simulink subsystem "pendulum_nonlinear"  (R2024b)
settings: Solver=VariableStepAuto  StartTime=0.0  StopTime=10.0  RelTol=1e-3
undefined symbols (not defined in the file): params
settings Model: Creator=dsagn  LastModifiedBy=dsagn
settings ModelReferenceCC: UpdateModelReferenceTargets=IfOutOfDate
settings SFSimCC: SimGPUStackLimitPerThread=51200
settings RTWCC: GPUStackLimitPerThread=51200  GPUComputeCapability=7.5
settings ConfigComp: CovMetricSettings=de  CovBoundaryAbsTol=1.0e-5

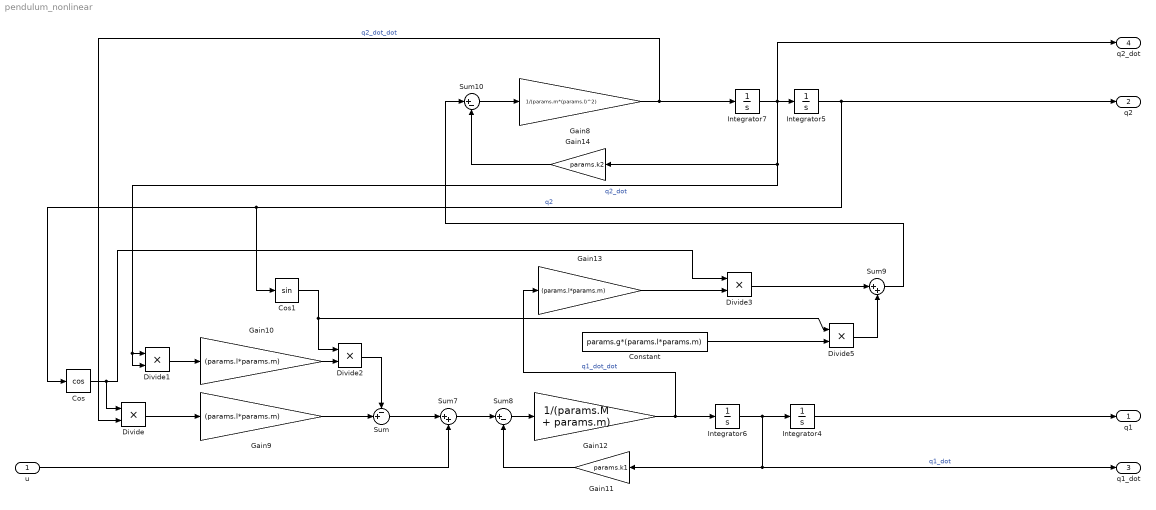
== system pendulum_nonlinear ==
  "u " : Inport
  Constant : Constant  Value=params.g*(params.l*params.m)
  Cos : Trigonometry  Operator=cos
  Cos1 : Trigonometry
  Divide{,1..3,5} (5 alike) : Product  Inputs=**
  Gain10 : Gain  Gain=(params.l*params.m)
  Gain11 : Gain  Gain=params.k1
  Gain12 : Gain  Gain=1/(params.M + params.m)
  Gain13 : Gain  Gain=(params.l*params.m)
  Gain14 : Gain  Gain=params.k2
  Gain8 : Gain  Gain=1/(params.m*(params.l)^2)
  Gain9 : Gain  Gain=(params.l*params.m)
  Integrator4 : Integrator  InitialCondition=params.IC(1)
  Integrator5 : Integrator  InitialCondition=params.IC(2)
  Integrator6 : Integrator  InitialCondition=params.IC(3)
  Integrator7 : Integrator  InitialCondition=params.IC(4)
  Sum : Sum  Inputs=-+|
  Sum10 : Sum  Inputs=|+-
  Sum7 : Sum  Inputs=|++
  Sum8 : Sum  Inputs=|+-
  Sum9 : Sum  Inputs=|++
  q1 : Outport  VectorParamsAs1DForOutWhenUnconnected=off
  "q2 " : Outport  Port=2  VectorParamsAs1DForOutWhenUnconnected=off
  q1_dot : Outport  Port=3  VectorParamsAs1DForOutWhenUnconnected=off
  q2_dot : Outport  Port=4  VectorParamsAs1DForOutWhenUnconnected=off
  wires:
  Sum7/1 -> Sum8/1
  Integrator7/1 -> Integrator5/1, Gain14/1, Divide1/1, Divide1/2, q2_dot/1  "q2_dot"
  Gain8/1 -> Integrator7/1, Divide/2  "q2_dot_dot"
  Gain14/1 -> Sum10/2
  Sum10/1 -> Gain8/1
  Integrator5/1 -> Cos/1, Cos1/1, "q2 "/1  "q2"
  Cos/1 -> Divide/1, Divide3/1
  Integrator6/1 -> Integrator4/1, Gain11/1, q1_dot/1  "q1_dot"
  Constant/1 -> Divide5/2
  Divide3/1 -> Sum9/1
  Sum/1 -> Sum7/1
  Sum9/1 -> Sum10/1
  Divide5/1 -> Sum9/2
  Divide/1 -> Gain9/1
  Gain9/1 -> Sum/2
  Sum8/1 -> Gain12/1
  Integrator4/1 -> q1/1
  "u "/1 -> Sum7/2
  Gain11/1 -> Sum8/2
  Gain13/1 -> Divide3/2
  Gain12/1 -> Integrator6/1, Gain13/1  "q1_dot_dot"
  Divide2/1 -> Sum/1
  Cos1/1 -> Divide5/1, Divide2/1
  Gain10/1 -> Divide2/2
  Divide1/1 -> Gain10/1
